simulink model "inverter"  (R2023b)
settings: Solver=VariableStepAuto  StartTime=0.0  StopTime=.1  RelTol=1e-3
libraries: spsIGBTLib x4, spsSeriesRLCBranchLib x4, spsCurrentMeasurementLib x2, spsFirstOrderFilterLib x2, spsACVoltageSourceLib x1, spsDCVoltageSourceLib x1, slpidlib x1, spsPLL3phLib x1, spsPLLLib x1, simulink x1, spsVoltageMeasurementLib x1, sps_lib x1
settings Model: Creator=ACER  LastModifiedBy=ACER
settings SolverCC: ZeroCrossAlgorithm=Adaptive
settings DataIOCC: SaveOutput=off  SignalLogging=off  DSMLogging=off  SaveTime=off  ReturnWorkspaceOutputs=off  LoggingToFile=on
settings DebuggingCC: IgnoredZcDiagnostic=none

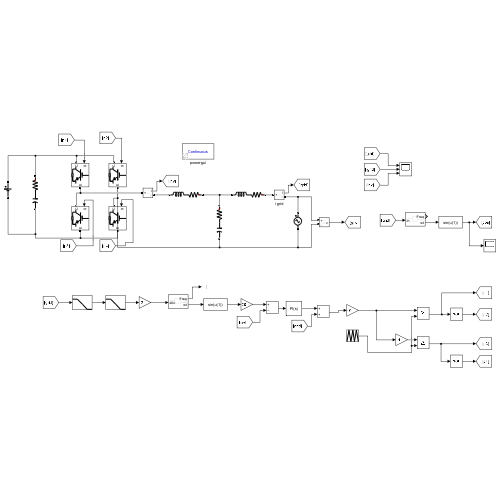
[thumbnail: Simulink's stored preview of the top-level diagram]
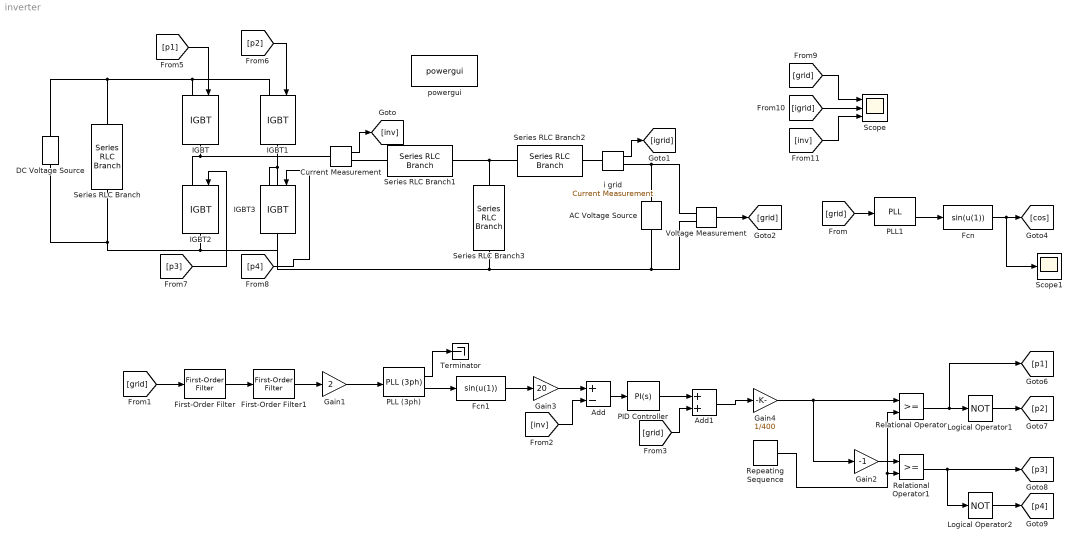
== system inverter ==
  AC Voltage Source : spsACVoltageSourceLib/AC Voltage Source  Amplitude=230*sqrt(2)  Phase=0  Frequency=50  SampleTime=0  Measurements=None  BusType=swing  Pref=10e3  Qref=0  Qmin=-inf  Qmax=+inf
  Add : Sum  Inputs=+-
  Add1 : Sum
  Current Measurement : spsCurrentMeasurementLib/Current Measurement  PhasorSimulation=off  OutputType=Complex  PSBequivalent=0
  DC Voltage Source : spsDCVoltageSourceLib/DC Voltage Source  Amplitude=400  Measurements=None
  Fcn : Fcn  Expr=sin(u(1))
  Fcn1 : Fcn  Expr=sin(u(1))
  First-Order Filter : spsFirstOrderFilterLib/First-Order Filter  FilterType=Lowpass  Tc=1/(2*pi*50)  Ts=0  Initialize=off  Vac_Init=[0, 0, 60]  Vdc_Init=0  PlotResponse=off  FreqRange="[0,  200,  1]"
  First-Order Filter1 : spsFirstOrderFilterLib/First-Order Filter  FilterType=Lowpass  Tc=1/(2*pi*50)  Ts=0  Initialize=off  Vac_Init=[0, 0, 60]  Vdc_Init=0  PlotResponse=off  FreqRange="[0,  200,  1]"
  Gain1 : Gain  Gain=2
  Gain2 : Gain  Gain=-1
  Gain3 : Gain  Gain=20
  Gain4 : Gain  Gain=1/400
  IGBT{,1..3} (4 alike) : spsIGBTLib/IGBT  Ron=0.001  Lon=0  Vf=1  Tf=1e-6  Tt=2e-6  IC=0  Rs=1e5  Cs=inf  Measurements=off
  Logical Operator1 : Logic  Operator=NOT  AllPortsSameDT=off  OutDataTypeStr=boolean
  Logical Operator2 : Logic  Operator=NOT  AllPortsSameDT=off  OutDataTypeStr=boolean
  PID Controller : slpidlib/PID Controller  Controller=PI  Form=Parallel  TimeDomain=Continuous-time  UseExternalTs=off  SampleTime=-1  IntegratorMethod=Forward Euler  FilterMethod=Forward Euler  ControllerParametersSource=internal  P=28  I=8  UseKiTs=off  D=0  N=100  UseFilter=on  TunerSelectOption=Transfer Function Based (PID Tuner App)  InitialConditionSource=internal  InitialConditionForIntegrator=0  InitialConditionForFilter=0  DifferentiatorICPrevScaledInput=0  ExternalReset=none  TrackingMode=off  Kt=1  LimitOutput=off  SatLimitsSource=internal  UpperSaturationLimit=inf  LowerSaturationLimit=-inf  LinearizeAsGain=on  AntiWindupMode=none  Kb=1  LimitIntegrator=off  UpperIntegratorSaturationLimit=inf  LowerIntegratorSaturationLimit=-inf  POutMin=[]  POutMax=[]  IOutMin=[]  IOutMax=[]  DOutMin=[]  DOutMax=[]  NOutMin=[]  NOutMax=[]  SumOutMin=[]  SumOutMax=[]  SaturationOutMin=[]  SaturationOutMax=[]  PParamMin=[]  PParamMax=[]  IParamMin=[]  IParamMax=[]  DParamMin=[]  DParamMax=[]  NParamMin=[]  NParamMax=[]  KbParamMin=[]  KbParamMax=[]  KtParamMin=[]  KtParamMax=[]  KbOutMin=[]  KbOutMax=[]  KtOutMin=[]  KtOutMax=[]  IntegratorOutMin=[]  IntegratorOutMax=[]  FilterOutMin=[]  FilterOutMax=[]  SumI1OutMin=[]  SumI1OutMax=[]  SumI2OutMin=[]  SumI2OutMax=[]  SumI3OutMin=[]  SumI3OutMax=[]  SumI4OutMin=[]  SumI4OutMax=[]  SumDOutMin=[]  SumDOutMax=[]  DifferentiatorOutMin=[]  DifferentiatorOutMax=[]  FilterDiffOutCoefMin=[]  FilterDiffOutCoefMax=[]  ReciprocalOutMin=[]  ReciprocalOutMax=[]  SumDenOutMin=[]  SumDenOutMax=[]  SumNumOutMin=[]  SumNumOutMax=[]  DivideOutMin=[]  DivideOutMax=[]  UdiffTsProdOutMin=[]  UdiffTsProdOutMax=[]  NTsProdOutMin=[]  NTsProdOutMax=[]  UintegralTsProdOutMin=[]  UintegralTsProdOutMax=[]  UngainTsProdOutMin=[]  UngainTsProdOutMax=[]  ClampingZeroOutDataTypeStr=Inherit: Inherit via back propagation  ClampingZeroOutMin=[]  ClampingZeroOutMax=[]  FilterDenConstantOutDataTypeStr=Inherit: Inherit via back propagation  FilterDenConstantOutMin=[]  FilterDenConstantOutMax=[]  PCopyOutDataTypeStr=Inherit: Inherit via back propagation  PCopyOutMin=[]  PCopyOutMax=[]  NCopyOutDataTypeStr=Inherit: Inherit via back propagation  NCopyOutMin=[]  NCopyOutMax=[]  IntegratorContinuousStateAttributes=''  IntegratorStateMustResolveToSignalObject=off  IntegratorRTWStateStorageClass=Auto  FilterContinuousStateAttributes=''  FilterStateMustResolveToSignalObject=off  FilterRTWStateStorageClass=Auto  ParallelPVariant=InternalParameters  IdealPVariant=Disabled  IVariant=InternalParameters  DVariant=Disabled  IntegratorVariant=Continuous  SatVariant=Disabled  AWVariant=Passthrough  PCopyVariant=Disabled  TRVariant=Disabled  FdbkBlocksVariant=Forward  IdealPFdbkVariant=Disabled  SatFdbkVariant=Disabled  DerivativeFilterVariant=Disabled  NVariant=Disabled  NCopyVariant=Disabled_SignalSpec  FilterICVariant=Disabled  IntegratorICVariant=InternalICs  ExternalResetVariant=Disabled  TRSumVariant=Passthrough  SumFdbkVariant=Disabled  SumVariant=Sum_PI  TsampFilterVariant=InternalTs  TsampNgainVariant=Passthrough  TsampIntegralVariant=Disabled_SignalSpec  ExternalSaturationOutDataTypeStr=Inherit: Same as second input
  PLL (3ph) : spsPLL3phLib/PLL (3ph)  Fmin=45  Par_Init=[0, 50]  ParK=[180, 3200, 1]  TcD=1e-4  MaxRateChangeFreq=12  FilterCutOffFreq=25  Ts=0  AGC=on
  PLL1 : spsPLLLib/PLL  Fmin=45  Par_Init=[0, 60]  ParK=[180, 3200, 1]  TcD=1e-4  MaxRateChangeFreq=12  FilterCutOffFreq=25  Ts=0  AGC=on
      settings: LibrarySourceBlock=sps_lib/Control/PLL
  Relational Operator : RelationalOperator  OutDataTypeStr=boolean  RndMeth=Simplest  InputSameDT=off
  Relational Operator1 : RelationalOperator  OutDataTypeStr=boolean  RndMeth=Simplest  InputSameDT=off
  Repeating Sequence : simulink/Sources/Repeating Sequence  rep_seq_t=[0 .00005 .0001]  rep_seq_y=[-1 1 -1]
  Scope : Scope  NumInputPorts=3
  Scope1 : Scope
  Series RLC Branch : spsSeriesRLCBranchLib/Series RLC Branch  LConnTagsString=__new0  RConnTagsString=__new0  BranchType=RC  Resistance=1e-3  Inductance=1e-3  SetiL0=off  InitialCurrent=0  Capacitance=500e-6  Setx0=off  InitialVoltage=0  Measurements=None
  Series RLC Branch1 : spsSeriesRLCBranchLib/Series RLC Branch  LConnTagsString=__new0  RConnTagsString=__new0  BranchType=RL  Resistance=.001  Inductance=4e-3  SetiL0=off  InitialCurrent=0  Capacitance=1e-6  Setx0=off  InitialVoltage=0  Measurements=None
  Series RLC Branch2 : spsSeriesRLCBranchLib/Series RLC Branch  LConnTagsString=__new0  RConnTagsString=__new0  BranchType=RL  Resistance=.0001  Inductance=4.15e-3  SetiL0=off  InitialCurrent=0  Capacitance=1e-6  Setx0=off  InitialVoltage=0  Measurements=None
  Series RLC Branch3 : spsSeriesRLCBranchLib/Series RLC Branch  LConnTagsString=__new0  RConnTagsString=__new0  BranchType=RC  Resistance=1e-3  Inductance=1e-3  SetiL0=off  InitialCurrent=0  Capacitance=2.2e-6  Setx0=off  InitialVoltage=0  Measurements=None
  Terminator : Terminator
  Voltage Measurement : spsVoltageMeasurementLib/Voltage Measurement  PhasorSimulation=off  OutputType=Complex  PSBequivalent=0
  i grid : spsCurrentMeasurementLib/Current Measurement  PhasorSimulation=off  OutputType=Complex  PSBequivalent=0
  powergui : sps_lib/powergui  Priority=1  SimulationMode=Continuous  SampleTime=50e-6  frequency=60  Iterations=50  frequencyindice=50  Pbase=100e6  ErrMax=1e-4  UnitsV=kV  UnitsW=MW  buscounter=0  FunctionMessages=off  echomessages=off  EnableUseOfTLC=off  CurrentSourceSwitches=off  DisableSnubberDevices=off  DisableRonSwitches=off  DisableVfSwitches=off  DisplayEquations=off  AutomaticDiscreteSolvers=off  SolverType=Tustin/Backward Euler (TBE)  Interpol=off  ExternalGateDelay=off  methode=off  Ts=100  x0status=blocks  SPID=on  SwTol=0  HookPort=off  NonlinearTolerance=1e-4  nMaxIteration=100  ContinueOnMaxIteration=off  RestoreLinks=warning  ResistiveCurrentMeasurement=off  Frange=[0:2:500]  Ylog=off  Xlog=on  ShowGrid=off  save=off  variable=ZData  structure=0  ZoomFFT=off  StartTime=0.0  cycles=1  DisplayStyle=1  fundamental=60  FreqAxis=off  MaxFrequency=1000  frequencyindicesteady=1  RmsSteady=1  display=off
  wires:
  Relational Operator/1 -> [p1], Logical Operator1/1
  [p1] -> IGBT/1
  [inv] -> Scope/3
  [grid] -> PLL1/1
  [grid] -> Scope/1
  Logical Operator2/1 -> [p4]
  Fcn/1 -> Scope1/1, [cos]
  Voltage Measurement/1 -> [grid]
  [p3] -> IGBT2/1
  Gain4/1 -> Gain2/1, Relational Operator/1
  Current Measurement/1 -> [inv]
  Gain2/1 -> Relational Operator1/1
  [p4] -> IGBT3/1
  [igrid] -> Scope/2
  [p2] -> IGBT1/1
  Repeating Sequence/1 -> Relational Operator/2, Relational Operator1/2
  PLL1/2 -> Fcn/1
  i grid/1 -> [igrid]
  Logical Operator1/1 -> [p2]
  Relational Operator1/1 -> [p3], Logical Operator2/1
  First-Order Filter/1 -> First-Order Filter1/1
  [grid] -> First-Order Filter/1
  First-Order Filter1/1 -> Gain1/1
  PLL (3ph)/2 -> Fcn1/1
  Fcn1/1 -> Gain3/1
  Gain1/1 -> PLL (3ph)/1
  Gain3/1 -> Add/1
  [inv] -> Add/2
  Add/1 -> PID Controller/1
  PID Controller/1 -> Add1/1
  [grid] -> Add1/2
  Add1/1 -> Gain4/1
  PLL (3ph)/1 -> Terminator/1
  connections:
  Series RLC Branch2/RConn1 -- Series RLC Branch1/LConn1 -- Series RLC Branch3/LConn1
  DC Voltage Source/LConn1 -- Series RLC Branch/RConn1 -- IGBT2/RConn1 -- IGBT3/RConn1
  AC Voltage Source/RConn1 -- Voltage Measurement/LConn1 -- i grid/RConn1
  DC Voltage Source/RConn1 -- Series RLC Branch/LConn1 -- IGBT1/LConn1 -- IGBT/LConn1
  Voltage Measurement/LConn2 -- AC Voltage Source/LConn1 -- Series RLC Branch3/RConn1 -- IGBT3/LConn1 -- IGBT1/RConn1
  Current Measurement/LConn1 -- IGBT2/LConn1 -- IGBT/RConn1
  Series RLC Branch1/RConn1 -- Current Measurement/RConn1
  i grid/LConn1 -- Series RLC Branch2/LConn1
